simulink model "Digital_Twin_of_EV_Drivetrain_Test_Rig"  (R2025a)
settings: Solver=ode23tb  StartTime=0.0  StopTime=inf  FixedStep=0.001  MaxStep=1e-3  RelTol=1e-3
PostLoadFcn:
  | , if any(exist('dsrtsu_mdlpostloadfcn', 'file') == [2, 3, 6]), try dsrtsu_mdlpostloadfcn('Execute', bdroot); catch fprintf('Error in PostLoadFcn (dsrtsu_mdlpostloadfcn) for model "%s":\n %s\n', bdroot, lasterr); end, end,
InitFcn:
  | , if any(exist('rtifpga_mdlclblib', 'file') ~= 0), rtifpga_mdlclblib('Init', bdroot); end,
values from neighbouring files (symbols this model uses):
  Af = 2.3    [Vehicle_Parameters.m]
  alpha = 0    [Vehicle_Parameters.m]
  Cd = 0.3    [Vehicle_Parameters.m]
  g = 9.81    [Vehicle_Parameters.m]
  Lambda = 1.05    [Vehicle_Parameters.m]
  M = 1600    [Vehicle_Parameters.m]
  r = 0.339    [Vehicle_Parameters.m]
  rho = 1.23    [Vehicle_Parameters.m]
  rrc = 0.01    [Vehicle_Parameters.m]
undefined symbols (not defined in the file or in its folder): acc, V
libraries: modbuslib x5, spsControlledVoltageSourceLib x3, simulink_extras x2, spsAsynchronousMachineSIUnitsLib x1, simulink x1, autolibshared x1, spsGroundLib x1, sps_lib x1
Description:
  | Standard RTI1202 template.
  | Supported MATLAB version:  R2024a.
settings Model: Tag=RTI1202  DSRTSU_INTERNAL_RTI_VER=650  DSRTSU_INTERNAL_RTI_TYPE=rti1202  RTICANMMDATA=struct('GeneralSetupData',struct('modelroot','C:\Users\VM-User\Desktop\MigrationScripts','generalsettings',struct('filesettings',struct('destfolder',struct('Name','RTICANMM_FILES','Check',1),'buildfolder',struct('Name','.','Check',1),'AbsDestfolder',struct('Name','C:\Users\VM-User\Desktop\MigrationScripts\RTICANMM_FILES'),'AbsBuildfolder',struct('Name','C:\Users\VM-User\Desktop\MigrationScripts'))),'options',struct('addpaths',1,'rmpaths',1,'addtrcexclusion',true,'cannavigator',struct('checkmonitoring',0),'show_usrtrc',0,'use_usrtrc',0),'advanced',struct('options',ones(1,100)),'MPSetup',{{}},'RTI',struct('Type','RTI1202','Ver','7.17','Date','02-Nov-2021'),'modelname','','block','untitled'))  DSRTSU_INTERNAL_RTIFPGA=210  DSRTSU_INTERNAL_RTISTBM_VER=24.2  Creator=24MLPC02  LastModifiedBy=nuhaa
settings SolverCC: AlgebraicLoopSolver=TrustRegion
settings DataIOCC: ReturnWorkspaceOutputs=off
settings OptimizationCC: BlockReduction=off  OptimizeBlockIOStorage=off  BufferReuse=off  ReuseModelBlockBuffer=off  GlobalBufferReuse=off  ExpressionFolding=off  LocalBlockOutputs=off  OptimizeDataStoreBuffers=off  BusAssignmentInplaceUpdate=off
settings DebuggingCC: UnconnectedInputMsg=warning  UnconnectedOutputMsg=warning  UnconnectedLineMsg=warning  PregeneratedLibrarySubsystemCodeDiagnostic=none  ArithmeticOperatorsInVariantConditions=warning
settings HardwareCC: ProdBitPerPointer=32.0  ProdBitPerSizeT=32.0  ProdBitPerPtrDiffT=32.0  ProdLargestAtomicInteger=Integer  ProdEndianess=BigEndian  ProdWordSize=32.0  ProdLongLongMode=on  ProdHWDeviceType=Custom Processor->Custom  TargetIntDivRoundTo=Zero  TargetEndianess=BigEndian  TargetHWDeviceType=Custom Processor->Custom
settings ModelReferenceCC: EnableRefExpFcnMdlSchedulingChecks=on  EnableParallelModelReferenceBuilds=on  ParallelModelReferenceMATLABWorkerInit=Load Top Model
settings SFSimCC: SimUseLocalCustomCode=off  MATLABDynamicMemAlloc=off  CustomCodeUndefinedFunction=UseInterfaceOnly
settings RTWCC: RTWUseLocalCustomCode=off  GPUComputeCapability=3.5  DLArmComputeVersion=19.05
settings CodeAppCC: StateflowObjectComments=on
settings GRTTargetCC: TargetLangStandard=C89/C90 (ANSI)
settings ConfigComp: CovMetricSettings=dswe

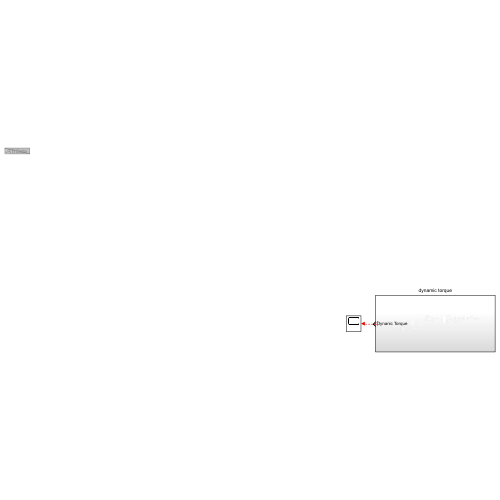
[thumbnail: Simulink's stored preview of the top-level diagram]
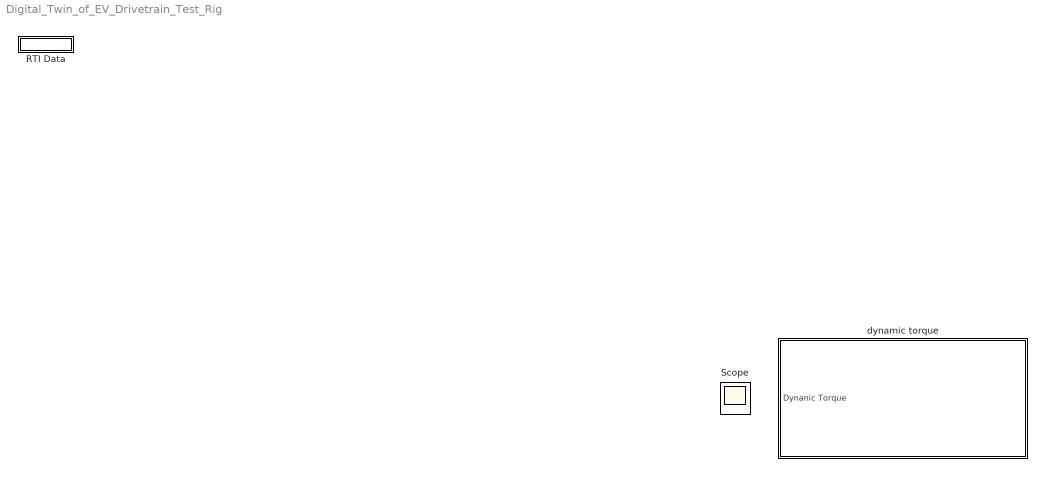
== system Digital_Twin_of_EV_Drivetrain_Test_Rig ==
  RTI Data : Subsystem  Tag=struct('RTIDataServer',struct('RTIDataServerVs','2','RTIModelDescription','struct(''main'',''Vehicle_dyna_admnuh'',''sub'',''Vehicle_dyna_admnuh'',''isMp'',0)'))  LoadFcn="if exist('rtidc'), try,  rtidc('DataHostBlockClbLoad', gcbh); catch, disp(['Warning: ''LoadFcn'' for RTI Data block failed: ' lasterr]); end, end,"  mask(RTI_DATA_HOST){}
      mask help:
      | RTI Data Block.
      | This block is used by RTI to store internal model-dependent data.
      | Please keep this block on the root level of the model. Deleting this block will result in data loss.
      |
      | NEVER DELETE OR COPY THIS BLOCK!
      settings: CopyFcn="if exist('rtidc'), try,  rtidc('DataHostBlockClbCopy', gcbh); catch, disp(['Warning: ''CopyFcn'' for RTI Data block failed: ' lasterr]); end, end,"  DeleteFcn="if exist('rtidc'), try,  rtidc('DataHostBlockClbDelete', gcbh); catch, disp(['Warning: ''DeleteFcn'' for RTI Data block failed: ' lasterr]); end, end,"  ModelCloseFcn="if exist('rtidc'), try,  rtidc('DataHostBlockClbModelClose', gcbh); catch, disp(['Warning: ''ModelCloseFcn'' for RTI Data block failed: ' lasterr]); end, end,"  PreSaveFcn="if exist('rtidc'), try,  rtidc('DataHostBlockClbPreSave', gcbh); catch, disp(['Warning: ''PreSaveFcn'' for RTI Data block failed: ' lasterr]); end, end,"  PostSaveFcn="if exist('rtidc'), try,  rtidc('DataHostBlockClbPostSave', gcbh); catch, disp(['Warning: ''PostSaveFcn'' for RTI Data block failed: ' lasterr]); end, end,"  NameChangeFcn="if exist('rtidc'), try,  rtidc('DataHostBlockClbNameChange', gcbh); catch, disp(['Warning: ''NameChangeFcn'' for RTI Data block failed: ' lasterr]); end, end,"
      mask Help:
      | RTI Data Block.
      | This block is used by RTI to store internal model-dependent data.
      | Please keep this block on the root level of the model. Deleting this block will result in data loss.
      | 
      | NEVER DELETE OR COPY THIS BLOCK!
      mask Display:
      | text(0.5, 0.5, 'RTI Data', 'HorizontalAlignment', 'center');
      | plot([1 0]);
  Scope : Scope
      settings: ActiveDisplayYMinimum=-1.2248012733282032  ActiveDisplayYMaximum=2.1864878870106916
  dynamic torque : Subsystem
  wires:
  ? -> Scope/1

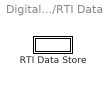
== system Digital_Twin_of_EV_Drivetrain_Test_Rig/RTI Data ==
  RTI Data Store : Subsystem  Tag=struct('private',struct('version',struct('dsVer',uint32(2)),'access',struct('type','Model','isPerm',1)))  mask(RTI_DATA_STORE){}
      mask help:
      | RTI Data Store Block. This block is used by RTI to store internal model dependent data. Deleting this block will result in data loss.
      |
      | NEVER DELETE, COPY, OR MODIFY THIS BLOCK!
      mask Help:
      | RTI Data Store Block. This block is used by RTI to store internal model dependent data. Deleting this block will result in data loss.
      | 
      | NEVER DELETE, COPY, OR MODIFY THIS BLOCK!
      mask Display: text(0.5, 0.5, ' ', 'HorizontalAlignment', 'center');

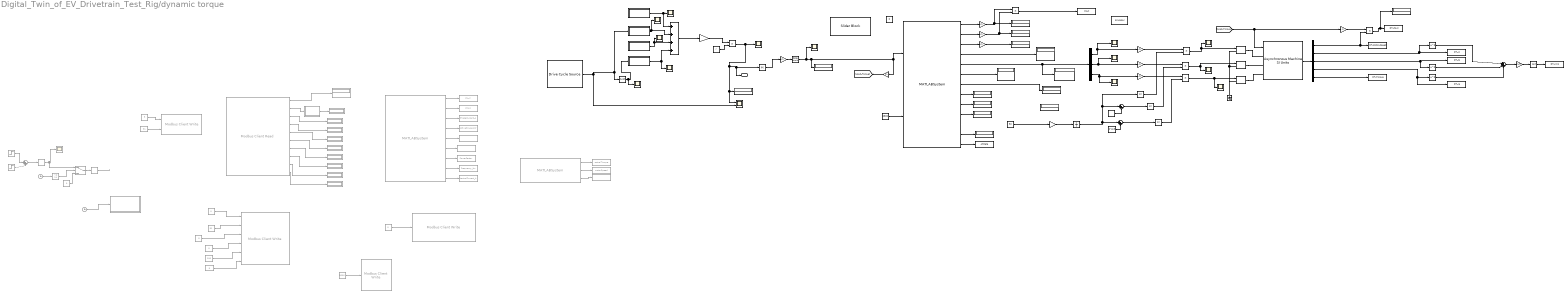
== system Digital_Twin_of_EV_Drivetrain_Test_Rig/dynamic torque ==
  Abs : Abs  SaturateOnIntegerOverflow=off
  Accelaration : Scope
      settings: ActiveDisplayYMinimum=-0.3125  ActiveDisplayYMaximum=2.8125  DataLoggingVariableName=ScopeData14
  Acceleration(inertia) Resistance : Subsystem
  Add : Sum  Inputs=++++
  Aerodynamic Drag : Subsystem
  Asynchronous Machine SI Units : spsAsynchronousMachineSIUnitsLib/Asynchronous Machine SI Units  RotorType=Squirrel-cage  PresetModel=No  MechanicalLoad=Torque Tm  ShowDetailedParameters=on  ReferenceFrame=Stationary  Units=SI  MeasurementBus=off  NominalParameters=[370 400 50]  VoltageRatio=1  Stator=[18.8 0.0561]  Rotor=[20.99 0.0561]  Cage1=[0.4155 0.002066]  Cage2=[0.4168 0.0003495]  Lm=1.45  Mechanical=[0.001 0.0006 1]  PolePairs=2  InitialConditions=[1 0 0 0 0 0 0 0]  SimulateSaturation=off  Saturation=[14.03593122, 27.81365428, 53.79336849, 72.68890987, 97.98006896, 148.6815601, 215.7428561, 302.9841135, 428.7778367 ; 230, 322, 414, 460, 506, 552, 598, 644, 690]  LoadFlowParameters=1492000  TsPowergui=0  TsBlock=-1  IterativeModel=Trapezoidal non iterative  IterativeDiscreteModel=Trapezoidal non iterative  Pmec=1.492e+006
  Bus Selector : BusSelector  OutputSignals=Mechanical.Rotor speed (wm),Stator measurements.Stator current is_c (A),Stator measurements.Stator current is_b (A),Stator measurements.Stator current is_a (A),Mechanical.Electromagnetic torque Te (N*m)
  Clock : Clock  Commented=on
  Clock2 : Clock  Commented=on
  Compare To Constant : simulink/Logic and Bit Operations/Compare To Constant  Commented=on  relop=<=  const=11  OutDataTypeStr=boolean
  Constant{,1,4,7} (4 alike) : Constant  Commented=on  Value=0
  Constant10 : Constant  Value=0
  Constant11 : Constant  Commented=on  Value=3000
  Constant12 : Constant  Value=50
  Constant13 : Constant  Commented=on  Value=31
  Constant15 : Constant  Value=2*pi/3
  Constant16 : Constant  Value=2*pi/3
  Constant2 : Constant  Commented=on  Value=51
  Constant3 : Constant  Commented=on  Value=5
  Constant5 : Constant  Commented=on  Value=100
  Constant6 : Constant  Commented=on  Value=5
  Constant8 : Constant  Value=2800
  Constant9 : Constant  Commented=on  Value=5
  Controlled Voltage Source : spsControlledVoltageSourceLib/Controlled Voltage Source  Initialize=on  Source_Type=AC  Amplitude=0  Phase=0  Frequency=0  Measurements=None
  Controlled Voltage Source1 : spsControlledVoltageSourceLib/Controlled Voltage Source  Initialize=on  Source_Type=AC  Amplitude=0  Phase=0  Frequency=0  Measurements=None
  Controlled Voltage Source2 : spsControlledVoltageSourceLib/Controlled Voltage Source  Initialize=on  Source_Type=AC  Amplitude=0  Phase=0  Frequency=0  Measurements=None
  Demux : Demux  Outputs=3
  Derivative : Derivative
  Display{,1..13} (14 alike) : Display
  Drive Cycle Source1 : autolibshared/Drive Cycle Source  cycleVar=US06  wsVar=driveCycle  fileVar=cycleFTP75.mat  tfinal="600  seconds"  cycleRepeat=off  outAccPort=off  outGearPort=off  gearList=No gear data  t_wot1=5  xdot_woto=0  xdot_wot1=30  t_wot2=20  xdot_wot2=0  t_wotend=30  srcUnit=m/s  outUnit=m/s  srcAccUnit=m/s/s  outAccUnit=m/s^2  dt=0  aMode=1  faultOption=off  velBnd=2  velBndUnit=mph  inUnit=m/s  timeBnd=1  failOption=off  stopSim=off  maxFaultCnt=10  maxFaultTime=2  maxTotFaultTime=15  traceOption=off  dtTrace=1  traceWindow=10  lastDCname=US06  lastOutUnit=mph  lastDT=0  lastTB=1  lastSB=2  forceCalcBound=off
  Gain : Gain  Gain=1/3
  Gain1 : Gain  Gain=-100/3.18
  Gain11 : Gain  Gain=-3.18/100
  Gain2 : Gain  Gain=sqrt(2)
  Gain3 : Gain  Gain=2*pi
  Gain4 : Gain  Gain=sqrt(2)
  Gain5 : Gain  Gain=sqrt(2)
  Gain6 : Gain  Gain=3.18/100
  Gain7 : Gain  Gain=-1
  Gain8 : Gain  Gain=3.18/100
  Gain9 : Gain  Gain=2*pi/60
  Gradient Resistance : Subsystem
  Ground : spsGroundLib/Ground  LConnTagsString=a
  Integrator : Integrator
  MATLAB Function : MATLAB Function  Commented=on  TreatAsAtomicUnit=on
  MATLAB Function1 : MATLAB Function  Commented=on  TreatAsAtomicUnit=on
  MATLAB System : MATLABSystem  Commented=on  System=ServoModbusIO  Port=COM7  BaudRate=38400  ServerID=1  SampleTime=0.1
      mask Type: ServoModbusIO
  MATLAB System1 : MATLABSystem  Commented=on  System=PowerMeterReader  Port=COM7  BaudRate=38400  ServerID=5  SampleTime=1
      mask Type: PowerMeterReader
  MATLAB System3 : MATLABSystem  System=DrivetrainModbusIO  Port=COM7  BaudRate=38400  SampleTime=0.1  InterTransactionDelay=0.015  RetryDelay=0.05  MaxModbusAttempts=3  MaxTorque_pct=50  MaxSpeed_rpm=2800  ServoID=6  PowerMeterID=3
      mask Type: DrivetrainModbusIO
  Modbus Client Read : modbuslib/Modbus Client Read  Commented=on  RetainClient=ModbusClient  ClientList=ModbusClient  ConnectionEndpoint=COM7  ServerId=1  RegisterTable={ '1', 'ActualTorque', '21', 'Holding Register', 'uint16', '2'; '2', 'ActualMotorSpeed', '19', 'Holding Register', 'uint16', '2'; '3', 'Speed&TorqueLimit(P1-02)', '261', 'Holding Register', 'uint16', '1'; '4', 'SpeedLimit(P1-55)', '367', 'Holding Register', 'uint16', '1'; '5', 'TorqueCommand(P1-12)', '281', 'Holding Register', 'uint16', '1'; '6', 'SONswitch(P4-07)', '1039', 'Holding Register', 'uint16', '1'; '7', 'DIcomm(P3-06)', '781', 'Holding Register', 'uint16', '1'; '8', 'ServoStatus(P0-46)', '93', 'Holding Register', 'uint16', '1'; '9', 'ServerID', '769', 'Holding Register', 'uint16', '1'; '10', 'speedLimit(P1-09)', '275', 'Holding Register', 'uint32', '1' }  SampleTime=1
  Modbus Client Write : modbuslib/Modbus Client Write  Commented=on  RetainClient=ModbusClient  ClientList=ModbusClient  ConnectionEndpoint=COM7  ServerId=2  RegisterTable={ '1', 'TorqueCommand(P1-12)', '281', 'Holding Register', 'int16'; '2', 'MonitorMethod', '35', 'Holding Register', 'uint16'; '3', 'SONswitch(P4-07)', '1039', 'Holding Register', 'uint16'; '4', 'SpeedLimitFn(P1-02)', '261', 'Holding Register', 'uint16'; '5', 'GlobalSpeedLimit(P1-55)', '367', 'Holding Register', 'uint16'; '6', 'DIcomm(P3-06)', '781', 'Holding Register', 'uint16' }  SampleTime=1
  Modbus Client Write1 : modbuslib/Modbus Client Write  Commented=on  RetainClient=ModbusClient  ClientList=ModbusClient  ConnectionEndpoint=COM7  ServerId=1  RegisterTable={ '1', 'TorqueCommand(P1-12)', '281', 'Holding Register', 'int16' }  SampleTime=1
  Modbus Client Write2 : modbuslib/Modbus Client Write  Commented=on  RetainClient=ModbusClient  ClientList=ModbusClient  ConnectionEndpoint=COM7  ServerId=2  RegisterTable={ '1', 'GlobalSpeedLimit(P1-55)', '367', 'Holding Register', 'uint16' }  SampleTime=1
  Modbus Client Write3 : modbuslib/Modbus Client Write  Commented=on  RetainClient=ModbusClient  ClientList=ModbusClient  ConnectionEndpoint=COM7  ServerId=1  RegisterTable={ '1', 'SONswitch(P4-07)', '1039', 'Holding Register', 'uint16'; '2', 'DIcomm(P3-06)', '781', 'Holding Register', 'uint16' }  SampleTime=1
  Product{1,3..7} (6 alike) : Product
  Rate Limiter : RateLimiter  RisingSlewLimit=10  FallingSlewLimit=-10  SampleTimeMode=inherited
  Read{,1..9} (10 alike) : Display  Commented=on
  Rolling Resistance Force : Subsystem
  Round : Rounding  Commented=on  Operator=round
  Round1 : Rounding  Commented=on  Operator=round
  Scale_down_factor2 : Gain  Gain=1/5000
  Scope{,3,6..9,12..17} (12 alike) : Scope
      Scope settings: ActiveDisplayYMinimum=-52.036405207705783  ActiveDisplayYMaximum=77.148137900648521
      Scope12 settings: ActiveDisplayYMinimum=-356.45169585110443  ActiveDisplayYMaximum=285.85050155134218  DataLoggingVariableName=ScopeData8
      Scope13 settings: DataLoggingVariableName=ScopeData9
      Scope14 settings: DataLoggingVariableName=ScopeData10
      Scope15 settings: ActiveDisplayYMinimum=-79.572460257694829  ActiveDisplayYMaximum=103.79630004184183  DataLoggingVariableName=ScopeData11
      Scope16 settings: ActiveDisplayYMinimum=-10.510942249240124  ActiveDisplayYMaximum=11.539057750759879  DataLoggingVariableName=ScopeData12
      Scope17 settings: ActiveDisplayYMinimum=45.17625  ActiveDisplayYMaximum=45.21375  DataLoggingVariableName=ScopeData13
      Scope3 settings: Title=Torque Vs Time  ActiveDisplayYMinimum=-0.44173938846228006  ActiveDisplayYMaximum=0.67264564769837742  DataLoggingVariableName=ScopeData7
      Scope6 settings: ActiveDisplayYMinimum=-4237.8652879640358  ActiveDisplayYMaximum=3608.1080500022067  DataLoggingVariableName=ScopeData15
      Scope7 settings: ActiveDisplayYMinimum=117.15430965827387  ActiveDisplayYMaximum=185.18984153315887  DataLoggingVariableName=ScopeData2
      Scope8 settings: ActiveDisplayYMinimum=-306.8845522858303  ActiveDisplayYMaximum=264.80141929224732  DataLoggingVariableName=ScopeData3
      Scope9 settings: ActiveDisplayYMinimum=-0.81263432505084165  ActiveDisplayYMaximum=0.83277062453292183  DataLoggingVariableName=ScopeData4
  Scope1 : Scope  NumInputPorts=2
      settings: ActiveDisplayYMinimum=-35.448988110084571  ActiveDisplayYMaximum=8.2107382667046771  DataLoggingVariableName=ScopeData5
  Scope4 : Scope  Commented=on
      settings: ActiveDisplayYMinimum=-0.56499977994060746  ActiveDisplayYMaximum=8.959188640297139  DataLoggingVariableName=ScopeData6
  Slider : SliderBlock  ScaleMin=-30  ScaleMax=30
  Sqrt : Sqrt
  Square : Math  Operator=square
  Square1 : Math  Operator=square
  Square2 : Math  Operator=square
  Step : Step  Commented=on  Time=2  After=5  SampleTime=0
  Step1 : Step  Commented=on  Time=10  After=-5  SampleTime=0
  Sum : Sum  Commented=on  Inputs=|++
  Sum1 : Sum  Inputs=|+-
  Sum2 : Sum  Inputs=|++
  Sum3 : Sum  Inputs=|+++
  Switch : Switch  Commented=on  Criteria=u2 > Threshold  SaturateOnIntegerOverflow=off  InputSameDT=off
  To Workspace : ToWorkspace  Commented=on  VariableName=actualTorque  SaveFormat=Timeseries  SampleTime=-1
  To Workspace1 : ToWorkspace  Commented=on  VariableName=motorSpeed  SaveFormat=Timeseries  SampleTime=-1
  To Workspace10 : ToWorkspace  VariableName=DT_Rotor_Speed  SaveFormat=Timeseries  SampleTime=-1
  To Workspace11 : ToWorkspace  VariableName=DT_Ic  SaveFormat=Timeseries  SampleTime=-1
  To Workspace12 : ToWorkspace  Commented=on  VariableName=Frequency_Hz  SaveFormat=Timeseries  SampleTime=-1
  To Workspace13 : ToWorkspace  VariableName=DT_Ib  SaveFormat=Timeseries  SampleTime=-1
  To Workspace14 : ToWorkspace  Commented=on  VariableName=NeutralCurrent_A  SaveFormat=Timeseries  SampleTime=-1
  To Workspace15 : ToWorkspace  VariableName=DT_Ia  SaveFormat=Timeseries  SampleTime=-1
  To Workspace16 : ToWorkspace  VariableName=DT_Torque  SaveFormat=Timeseries  SampleTime=-1
  To Workspace17 : ToWorkspace  VariableName=DT_Pout  SaveFormat=Timeseries  SampleTime=-1
  To Workspace18 : ToWorkspace  VariableName=Pout  SaveFormat=Timeseries  SampleTime=-1
  To Workspace19 : ToWorkspace  VariableName=DT_Irms  SaveFormat=Timeseries  SampleTime=-1
  To Workspace2 : ToWorkspace  Commented=on  VariableName=CommandTorquePCT  SaveFormat=Timeseries  SampleTime=-1
  To Workspace24 : ToWorkspace  VariableName=AllData  SaveFormat=Timeseries  SampleTime=-1
  To Workspace3 : ToWorkspace  Commented=on  VariableName=VLL_V  SaveFormat=Timeseries  SampleTime=-1
  To Workspace4 : ToWorkspace  Commented=on  VariableName=VLN_V  SaveFormat=Timeseries  SampleTime=-1
  To Workspace5 : ToWorkspace  Commented=on  VariableName=PhaseCurrent_A  SaveFormat=Timeseries  SampleTime=-1
  To Workspace6 : ToWorkspace  Commented=on  VariableName=ActivePower_kW  SaveFormat=Timeseries  SampleTime=-1
  To Workspace7 : ToWorkspace  Commented=on  VariableName=ApparentPower_kVA  SaveFormat=Timeseries  SampleTime=-1
  To Workspace8 : ToWorkspace  Commented=on  VariableName=ReactivePower_kVAr  SaveFormat=Timeseries  SampleTime=-1
  To Workspace9 : ToWorkspace  Commented=on  VariableName=PowerFactor  SaveFormat=Timeseries  SampleTime=-1
  Torque(Nm) : Display
  Trigonometric Function : Trigonometry
  Trigonometric Function1 : Trigonometry
  Trigonometric Function2 : Trigonometry
  Wheel Radius : Constant  Value=r
  powergui1 : sps_lib/powergui  Priority=1  SimulationMode=Continuous  SampleTime=50e-6  frequency=60  Iterations=50  frequencyindice=50  Pbase=100e6  ErrMax=1e-4  UnitsV=kV  UnitsW=MW  buscounter=0  FunctionMessages=off  echomessages=off  EnableUseOfTLC=off  CurrentSourceSwitches=off  DisableSnubberDevices=off  DisableRonSwitches=off  DisableVfSwitches=off  DisplayEquations=off  AutomaticDiscreteSolvers=off  SolverType=Tustin/Backward Euler (TBE)  Interpol=off  ExternalGateDelay=off  methode=off  Ts=100  x0status=blocks  SPID=on  SwTol=0  HookPort=off  NonlinearTolerance=1e-4  nMaxIteration=100  ContinueOnMaxIteration=off  RestoreLinks=warning  ResistiveCurrentMeasurement=off  Frange=[0:2:500]  Ylog=off  Xlog=on  ShowGrid=off  save=off  variable=ZData  structure=0  ZoomFFT=off  StartTime=0.0  cycles=1  DisplayStyle=1  fundamental=60  FreqAxis=off  MaxFrequency=1000  frequencyindicesteady=1  RmsSteady=1  display=off
  Dynanic Torque : Outport
  wires:
  Modbus Client Read/1 -> Read/1
  Modbus Client Read/2 -> MATLAB Function/1(v)
  Constant2/1 -> Modbus Client Write/2
  MATLAB Function/1(rpm) -> Read1/1
  Modbus Client Read/3 -> Read2/1
  Modbus Client Read/4 -> Read3/1
  Modbus Client Read/5 -> Read4/1
  Modbus Client Read/6 -> Read5/1
  Constant1/1 -> Modbus Client Write/1
  Constant3/1 -> Modbus Client Write/3
  Constant4/1 -> Modbus Client Write/4
  Constant5/1 -> Modbus Client Write/5
  Modbus Client Read/7 -> Read6/1
  Constant6/1 -> Modbus Client Write/6
  Constant11/1 -> Modbus Client Write2/1
  Modbus Client Read/8 -> Read7/1
  MATLAB System/3 -> To Workspace2/1
  MATLAB System/2 -> To Workspace1/1
  MATLAB System/1 -> To Workspace/1
  Modbus Client Read/9 -> Read8/1
  MATLAB System1/1 -> To Workspace3/1
  MATLAB System1/2 -> To Workspace4/1
  MATLAB System1/3 -> To Workspace5/1
  MATLAB System1/4 -> To Workspace6/1
  MATLAB System1/7 -> To Workspace9/1
  MATLAB System1/9 -> To Workspace14/1
  MATLAB System1/6 -> To Workspace7/1
  MATLAB System1/5 -> To Workspace8/1
  MATLAB System1/8 -> To Workspace12/1
  Modbus Client Read/10 -> Read9/1
  Constant8/1 -> MATLAB System3/2
  Switch/1 -> Round1/1
  Round/1 -> Switch/1, Scope4/1
  Step1/1 -> Sum/2
  Clock/1 -> Compare To Constant/1
  Sum/1 -> Round/1
  Constant7/1 -> Switch/3
  Step/1 -> Sum/1
  Round1/1 -> ?
  Compare To Constant/1 -> Switch/2
  MATLAB System3/1 -> Gain8/1
  MATLAB System3/2 -> Gain9/1
  MATLAB System3/3 -> Gain6/1
  MATLAB System3/5 -> Demux/1, Display4/1
  MATLAB System3/6 -> Display5/1
  MATLAB System3/7 -> Display6/1
  MATLAB System3/8 -> Display7/1
  MATLAB System3/9 -> Display8/1
  MATLAB System3/10 -> Display9/1
  Gain3/1 -> Integrator/1
  Demux/2 -> Scope16/1, Gain4/1
  Demux/1 -> Gain2/1, Scope15/1
  Gain2/1 -> Product3/1
  Trigonometric Function/1 -> Product3/2
  Constant15/1 -> Sum1/2
  Sum1/1 -> Trigonometric Function1/1
  Trigonometric Function1/1 -> Product4/2
  Gain4/1 -> Product4/1
  Constant16/1 -> Sum2/2
  Sum2/1 -> Trigonometric Function2/1
  Trigonometric Function2/1 -> Product5/2
  Gain5/1 -> Product5/1
  Product5/1 -> Scope14/1, Controlled Voltage Source2/1
  Product4/1 -> Controlled Voltage Source1/1, Scope13/1
  Product3/1 -> Scope12/1, Controlled Voltage Source/1
  Asynchronous Machine SI Units/1 -> Bus Selector/1
  Bus Selector/1 -> Product6/2, To Workspace10/1  "<Rotor speed (wm)>"
  Bus Selector/2 -> Square/1, To Workspace11/1  "<Stator current is_c (A)>"
  Bus Selector/3 -> Square1/1, To Workspace13/1  "<Stator current is_b (A)>"
  Bus Selector/4 -> To Workspace15/1, Square2/1  "<Stator current is_a (A)>"
  Bus Selector/5 -> To Workspace16/1  "<Electromagnetic torque Te (N*m)>"
  Demux/3 -> Scope17/1, Gain5/1
  MATLAB System3/13 -> To Workspace24/1
  Gain6/1 -> Display2/1
  Gain8/1 -> Display/1, Product7/1
  MATLAB System3/12 -> Display11/1
  Product6/1 -> Display12/1, To Workspace17/1
  Product7/1 -> To Workspace18/1
  Gain9/1 -> Product7/2, Display1/1
  Constant13/1 -> Modbus Client Write3/2
  Constant9/1 -> Modbus Client Write3/1
  Constant/1 -> Modbus Client Write1/1
  Clock2/1 -> MATLAB Function1/1(t)
  MATLAB System3/4 -> Display13/1
  [Load_Torque] -> Gain7/1, Asynchronous Machine SI Units/1
  Gain7/1 -> Product6/1
  Derivative/1 -> Accelaration/1, Acceleration(inertia) Resistance/1(Acceleration)
  Wheel Radius/1 -> Product1/2
  Add/1 -> Scale_down_factor2/1
  Rolling Resistance Force/1(Frr) -> Add/1, Scope7/1
  Gain1/1 -> Rate Limiter/1
  Drive Cycle Source1/1 -> Scope1/2, Derivative/1, Aerodynamic Drag/1(V(m/s))
  Gradient Resistance/1(Fgr) -> Scope9/1, Add/3
  Aerodynamic Drag/1(Fad) -> Scope8/1, Add/2
  Scale_down_factor2/1 -> Product1/1
  Abs/1 -> Gain1/1
  Acceleration(inertia) Resistance/1(Fa) -> Scope6/1, Add/4
  Product1/1 -> Abs/1, Dynanic Torque/1, Scope1/1, Torque(Nm)/1, Scope3/1
  Rate Limiter/1 -> Scope/1, MATLAB System3/1, Gain11/1, Display3/1
  Sum3/1 -> Gain/1
  Gain/1 -> Sqrt/1
  Sqrt/1 -> To Workspace19/1
  Square/1 -> Sum3/1
  Square2/1 -> Sum3/3
  Square1/1 -> Sum3/2
  Integrator/1 -> Sum2/1, Trigonometric Function/1, Sum1/1
  Constant12/1 -> Gain3/1
  Gain11/1 -> [Load_Torque]
  connections:
  Controlled Voltage Source/RConn1 -- Asynchronous Machine SI Units/LConn1
  Controlled Voltage Source1/RConn1 -- Asynchronous Machine SI Units/LConn2
  Controlled Voltage Source2/RConn1 -- Asynchronous Machine SI Units/LConn3
  Controlled Voltage Source/LConn1 -- Ground/LConn1 -- Controlled Voltage Source2/LConn1 -- Controlled Voltage Source1/LConn1

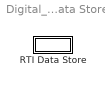
== system Digital_Twin_of_EV_Drivetrain_Test_Rig/RTI Data/RTI Data Store ==
  RTI Data Store : Subsystem  mask(RTI_DATA_STORE){}
      mask help:
      | RTI Data Store Block. This block is used by RTI to store internal model dependent data. Deleting this block will result in data loss.
      |
      | NEVER DELETE, COPY, OR MODIFY THIS BLOCK!
      mask Help:
      | RTI Data Store Block. This block is used by RTI to store internal model dependent data. Deleting this block will result in data loss.
      | 
      | NEVER DELETE, COPY, OR MODIFY THIS BLOCK!
      mask Display: text(0.5, 0.5, ' ', 'HorizontalAlignment', 'center');

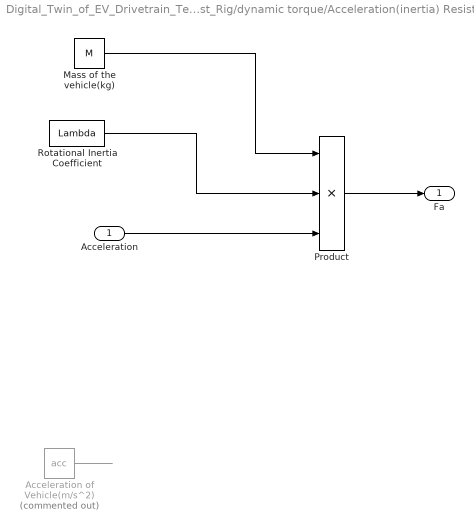
== system Digital_Twin_of_EV_Drivetrain_Test_Rig/dynamic torque/Acceleration(inertia) Resistance ==
  Acceleration : Inport
  Acceleration of Vehicle(m/s^2) : Constant  Commented=on  Value=acc
  Mass of the vehicle(kg) : Constant  Value=M
  Product : Product  Inputs=3
  Rotational Inertia Coefficient : Constant  Value=Lambda
  Fa : Outport
  wires:
  Mass of the vehicle(kg)/1 -> Product/1
  Acceleration of Vehicle(m/s^2)/1 -> ?
  Rotational Inertia Coefficient/1 -> Product/2
  Product/1 -> Fa/1
  Acceleration/1 -> Product/3

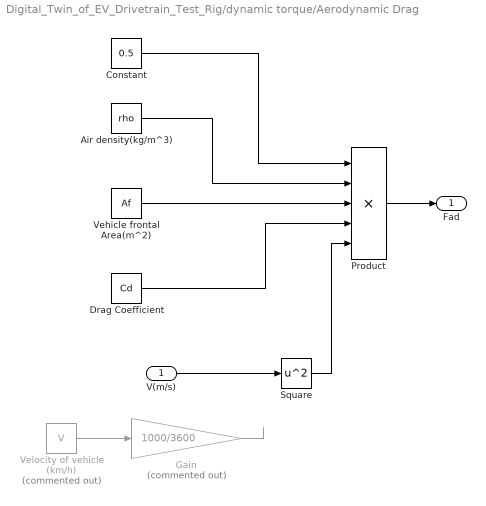
== system Digital_Twin_of_EV_Drivetrain_Test_Rig/dynamic torque/Aerodynamic Drag ==
  V(m/s) : Inport
  Air density(kg/m^3) : Constant  Value=rho
  Constant : Constant  Value=0.5
  Drag Coefficient : Constant  Value=Cd
  Gain : Gain  Commented=on  Gain=1000/3600
  Product : Product  Inputs=5
  Square : Math  Operator=square
  Vehicle frontal Area(m^2) : Constant  Value=Af
  Velocity of vehicle (km/h) : Constant  Commented=on  Value=V
  Fad : Outport
  wires:
  Velocity of vehicle (km/h)/1 -> Gain/1
  Gain/1 -> ?
  Constant/1 -> Product/1
  Air density(kg/m^3)/1 -> Product/2
  Vehicle frontal Area(m^2)/1 -> Product/3
  Drag Coefficient/1 -> Product/4
  Square/1 -> Product/5
  Product/1 -> Fad/1
  V(m/s)/1 -> Square/1

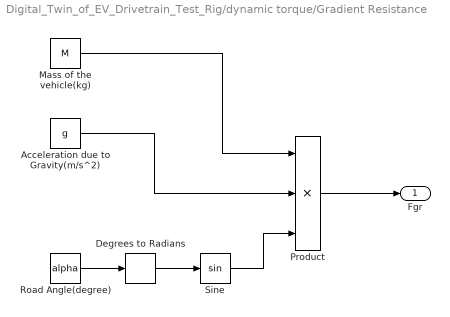
== system Digital_Twin_of_EV_Drivetrain_Test_Rig/dynamic torque/Gradient Resistance ==
  Acceleration due to Gravity(m/s^2) : Constant  Value=g
  Degrees to Radians : simulink_extras/Transformations/Degrees to Radians
  Mass of the vehicle(kg) : Constant  Value=M
  Product : Product  Inputs=3
  Road Angle(degree) : Constant  Value=alpha
  Sine : Trigonometry
  Fgr : Outport
  wires:
  Mass of the vehicle(kg)/1 -> Product/1
  Road Angle(degree)/1 -> Degrees to Radians/1
  Acceleration due to Gravity(m/s^2)/1 -> Product/2
  Degrees to Radians/1 -> Sine/1
  Product/1 -> Fgr/1
  Sine/1 -> Product/3

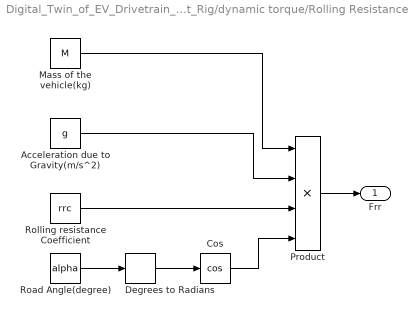
== system Digital_Twin_of_EV_Drivetrain_Test_Rig/dynamic torque/Rolling Resistance Force ==
  Acceleration due to Gravity(m/s^2) : Constant  Value=g
  Cos : Trigonometry  Operator=cos
  Degrees to Radians : simulink_extras/Transformations/Degrees to Radians
  Mass of the vehicle(kg) : Constant  Value=M
  Product : Product  Inputs=4
  Road Angle(degree) : Constant  Value=alpha
  Rolling resistance Coefficient : Constant  Value=rrc
  Frr : Outport
  wires:
  Road Angle(degree)/1 -> Degrees to Radians/1
  Degrees to Radians/1 -> Cos/1
  Mass of the vehicle(kg)/1 -> Product/1
  Acceleration due to Gravity(m/s^2)/1 -> Product/2
  Rolling resistance Coefficient/1 -> Product/3
  Cos/1 -> Product/4
  Product/1 -> Frr/1

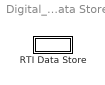
== system Digital_Twin_of_EV_Drivetrain_Test_Rig/RTI Data/RTI Data Store/RTI Data Store ==
  RTI Data Store : Subsystem  mask(RTI_DATA_STORE){}
      mask help:
      | RTI Data Store Block. This block is used by RTI to store internal model dependent data. Deleting this block will result in data loss.
      |
      | NEVER DELETE, COPY, OR MODIFY THIS BLOCK!
      mask Help:
      | RTI Data Store Block. This block is used by RTI to store internal model dependent data. Deleting this block will result in data loss.
      | 
      | NEVER DELETE, COPY, OR MODIFY THIS BLOCK!
      mask Display: text(0.5, 0.5, ' ', 'HorizontalAlignment', 'center');

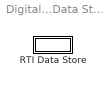
== system Digital_Twin_of_EV_Drivetrain_Test_Rig/RTI Data/RTI Data Store/RTI Data Store/RTI Data Store ==
  RTI Data Store : Subsystem  mask(RTI_DATA_STORE){}
      mask help:
      | RTI Data Store Block. This block is used by RTI to store internal model dependent data. Deleting this block will result in data loss.
      |
      | NEVER DELETE, COPY, OR MODIFY THIS BLOCK!
      mask Help:
      | RTI Data Store Block. This block is used by RTI to store internal model dependent data. Deleting this block will result in data loss.
      | 
      | NEVER DELETE, COPY, OR MODIFY THIS BLOCK!
      mask Display: text(0.5, 0.5, ' ', 'HorizontalAlignment', 'center');

== system Digital_Twin_of_EV_Drivetrain_Test_Rig/RTI Data/RTI Data Store/RTI Data Store/RTI Data Store/RTI Data Store ==

== matlab function Digital_Twin_of_EV_Drivetrain_Test_Rig/dynamic torque/MATLAB Function ==
  data: v input double size=[1 2]; rpm output double size=[1 1]
function rpm = decodeSpeed(v)

lo = uint32(v(1));
hi = uint32(v(2));

raw = bitor(lo, bitshift(hi,16));

if raw >= uint32(2147483648)
    signedValue = double(raw) - 4294967296;
else
    signedValue = double(raw);
end

rpm = signedValue / 10;

== matlab function Digital_Twin_of_EV_Drivetrain_Test_Rig/dynamic torque/MATLAB Function1 ==
  data: t input; TorqueCmd_pct output
function TorqueCmd_pct = TrapezoidTorque(t)

% Trapezium torque settings
Tmax = 4;      % Maximum commanded torque (%)

t1 = 2;         % Start ramp-up
t2 = 5;         % End ramp-up
t3 = 10;        % Start ramp-down
t4 = 13;        % End ramp-down

% Generate trapezium
if t < t1

    TorqueCmd_pct = 0;

elseif t < t2

    % Ramp from 0 to Tmax
    TorqueCmd_pct = Tmax * (t - t1)/(t2 - t1);

elseif t < t3

    % Hold Tmax
    TorqueCmd_pct = Tmax;

elseif t < t4

    % Ramp from Tmax back to zero
    TorqueCmd_pct = Tmax * ...
        (1 - (t - t3)/(t4 - t3));

else

    TorqueCmd_pct = 0;

end
